simulink model "DCHR_A44_Graphical_Supervisor"  (R2026a)
settings: Solver=FixedStepDiscrete  StopTime=603900  FixedStep=900
settings Model: Creator=Lysda  LastModifiedBy=Lysda

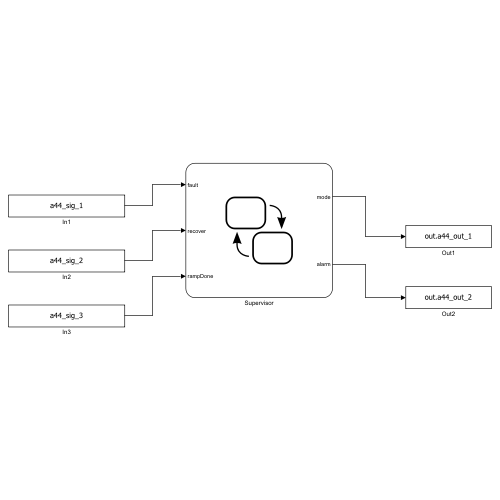
[thumbnail: Simulink's stored preview of the top-level diagram]
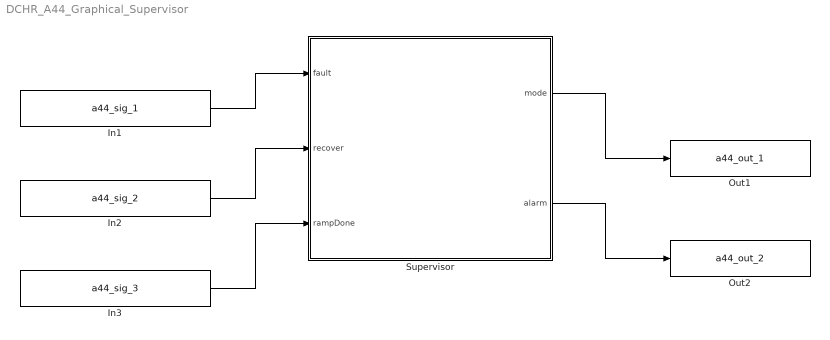
== system DCHR_A44_Graphical_Supervisor ==
  In1 : FromWorkspace  VariableName=a44_sig_1
  In2 : FromWorkspace  VariableName=a44_sig_2
  In3 : FromWorkspace  VariableName=a44_sig_3
  Out1 : ToWorkspace  VariableName=a44_out_1  SampleTime=-1
  Out2 : ToWorkspace  VariableName=a44_out_2  SampleTime=-1
  Supervisor : Stateflow chart  TreatAsAtomicUnit=on
  wires:
  In1/1 -> Supervisor/1(fault)
  In2/1 -> Supervisor/2(recover)
  In3/1 -> Supervisor/3(rampDone)
  Supervisor/1(mode) -> Out1/1
  Supervisor/2(alarm) -> Out2/1

== stateflow chart DCHR_A44_Graphical_Supervisor/Supervisor ==
  state ACTIVE
    entry: mode=0; alarm=0;
  state TRIP_PENDING
    entry: mode=1; alarm=1; pending=1;
    during: pending=pending+1;
  state RAMPING
    entry: mode=3; alarm=1;
  state TRIPPED
    entry: mode=2; alarm=2; good=0;
    during: if recover && ~fault; good=good+1; else; good=0; end
  TRIP_PENDING -> ACTIVE [order 1] : [~fault && recover]
  (default) -> ACTIVE
  RAMPING -> ACTIVE [order 1] : [rampDone && ~fault]
  RAMPING -> TRIP_PENDING [order 2] : [fault]
  ACTIVE -> TRIP_PENDING : [fault]
  TRIP_PENDING -> TRIPPED [order 2] : [pending>=2]
  TRIPPED -> RAMPING : [good>=1 && recover && ~fault]
  data: fault input; recover input; rampDone input; mode output; alarm output; pending local; good local
